simulink model "test1"  (R2025b)
settings: Solver=VariableStepAuto  StartTime=0.0  StopTime=10.0  MaxStep=0.01  RelTol=1e-3
settings Model: Creator=Shriram  LastModifiedBy=Shriram

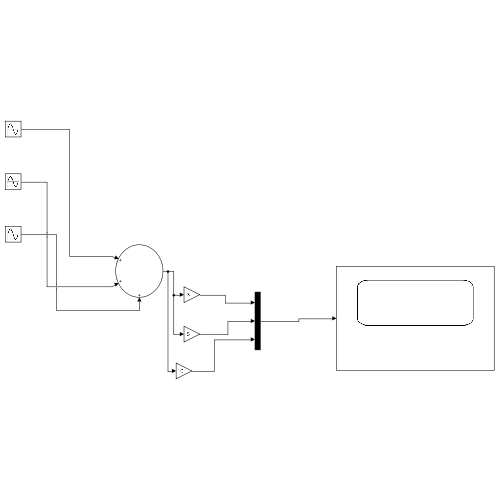
[thumbnail: Simulink's stored preview of the top-level diagram]
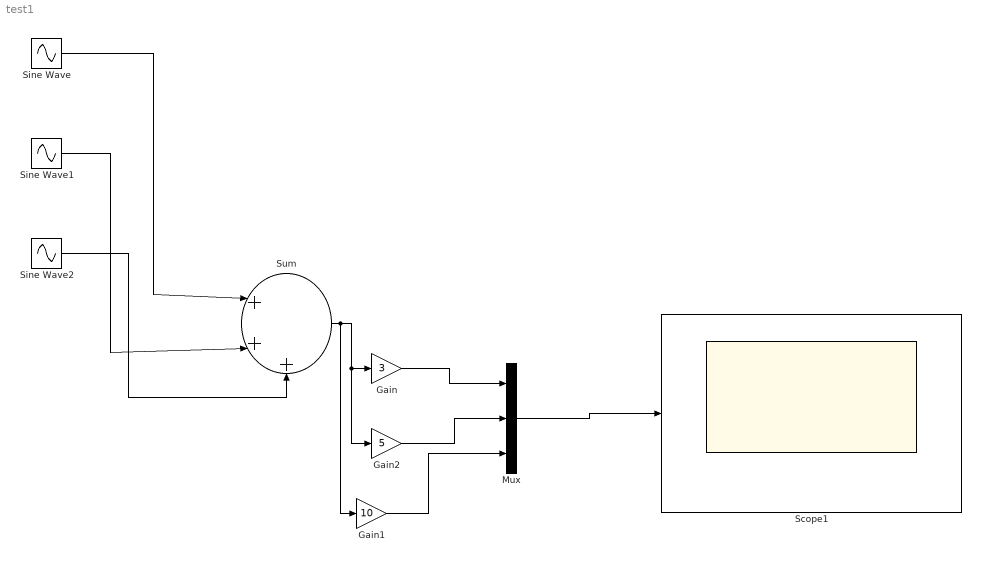
== system test1 ==
  Gain : Gain  Gain=3
  Gain1 : Gain  Gain=10
  Gain2 : Gain  Gain=5
  Mux : Mux  Inputs=3
  Scope1 : Scope
      settings: ActiveDisplayYMinimum=-34.400175950066789  ActiveDisplayYMaximum=34.399800198065613
  Sine Wave : Sin  SampleTime=0
  Sine Wave1 : Sin  Frequency=5  SampleTime=0
  Sine Wave2 : Sin  Frequency=10  SampleTime=0
  Sum : Sum  Inputs=|+++
  wires:
  Sine Wave/1 -> Sum/1
  Sine Wave1/1 -> Sum/2
  Sine Wave2/1 -> Sum/3
  Sum/1 -> Gain1/1, Gain2/1, Gain/1
  Gain/1 -> Mux/1
  Gain2/1 -> Mux/2
  Gain1/1 -> Mux/3
  Mux/1 -> Scope1/1
